simulink model "SarAdc"  (R2024a)
settings: Solver=VariableStepDiscrete  StartTime=0  StopTime=P.stop_time_s  RelTol=1e-3
PostLoadFcn:
  | addpath(genpath(fullfile(fileparts(fileparts(get_param(bdroot,'FileName'))),'src')),'-begin');
InitFcn:
  | addpath(genpath(fullfile(fileparts(fileparts(get_param(bdroot,'FileName'))),'src')),'-begin');
model workspace (MAT data in the model file):
  DecodeP.schema = 'sar20-behavior-decode/v1'
  DecodeP.vref_v = 5
  DecodeP.fsr_diff_v = 10
  DecodeP.ra_gain = 32
  DecodeP.d2_weights_ra_v = [0.36; 0.24; 0.16; 0.104; 0.064; 0.04; 0.024; 0.012; 0.008; 0.004; 0.002; 0.001]
  DecodeP.d2_offset_ra_v = -0.5095
  DecodeP.tracking_step_ra_v = 0.00025
  DecodeP.dither_enabled = 0
  DecodeP.dither_seed = 20261223
  DecodeP.dither_amplitude_v = 0.001
  DecodeP.calibration_mode = 'off'
  DecodeP.tracking_mode = 'finite_sinc2'
  DecodeP.az_mode = 'ordinary'
  DecodeP.coefficient_source = 'nominal saved.fpga weights only; new DAC1 geometry formula'
  DecodeP.d1_bias_v = 0
  P : object (value not decoded)
  TrainCaptureFile = ''
symbols that are objects in the model workspace (value not decoded): P
undefined symbols (not defined in the file): sar20_pp_initial_state, sar20_pp_verified_parameters
settings Model: Creator=Administrator  LastModifiedBy=Administrator
settings DataIOCC: SignalLogging=off

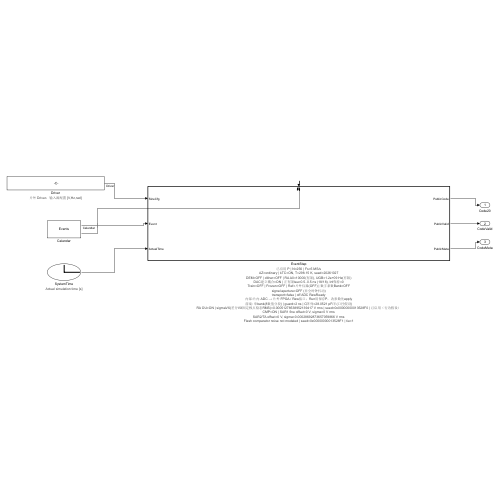
[thumbnail: Simulink's stored preview of the top-level diagram]
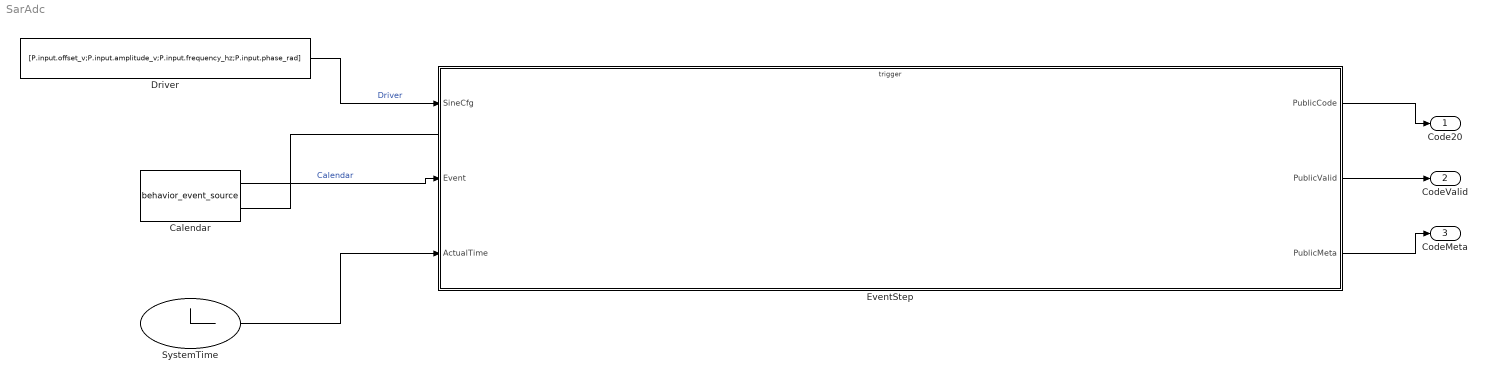
== system SarAdc ==
  Calendar : M-S-Function  FunctionName=behavior_event_source  Parameters=P.schedule
      mask Display: disp('Events')
  Driver : Constant  Value=[P.input.offset_v;P.input.amplitude_v;P.input.frequency_hz;P.input.phase_rad]
      settings: AttributesFormatString=片外 Driver：输入源配置 [V,Hz,rad]
  EventStep : Subsystem
      settings: AttributesFormatString=|
      | 已应用 P | N=256 | Fs=5 MS/s
      | AZ=ordinary | kTC=ON, T=298.15 K, seed=20261027
      | DEM=OFF | dither=OFF | RA A0=10000(有限), UGB=1.2e+09 Hz(有限)
      | DAC建立耦合=ON | 正有限tau=0.5..0.5 ns (18/18), Inf保持=0
      | Train=OFF | Frozen=OFF | Ref=片外仪器(OFF) | 数字系数Bank=OFF
      | signal aperture=OFF (非全时钟抖动)
      | transport=false | off ADC RawReady
      | 内部:片内 ADC → 片外 FPGA / Raw接口；Run用保存P，改参数先apply
      | 前端: 单bank(8数值分段) | guard=2 ns | C阵列=28.0521 pF/半(口径假设)
      | RA OU=ON | sigmaVX(差分VX固定极点稳态RMS)=0.00051278538952139417 V rms | seed=0x00000000013528F0 | 已启用（行为假设）
      | CMP=ON | SAR1 fine offset=0 V, sigma=0 V rms
      | SAR2/TA offset=0 V, sigma=0.00028692873657059866 V rms
      | Flash comparator noise not modeled | seed=0x00000000013528F1 | tie=1
  SystemTime : Clock
      settings: AttributesFormatString=Actual simulation time [s]
  Code20 : Outport  PortDimensions=1
  CodeValid : Outport  Port=2  PortDimensions=1
  CodeMeta : Outport  Port=3  PortDimensions=9
  wires:
  EventStep/3(PublicMeta) -> CodeMeta/1
  EventStep/2(PublicValid) -> CodeValid/1
  EventStep/1(PublicCode) -> Code20/1
  SystemTime/1 -> EventStep/3(ActualTime)
  Calendar/2 -> EventStep/Trigger
  Driver/1 -> EventStep/1(SineCfg)  "Driver"
  Calendar/1 -> EventStep/2(Event)  "Calendar"

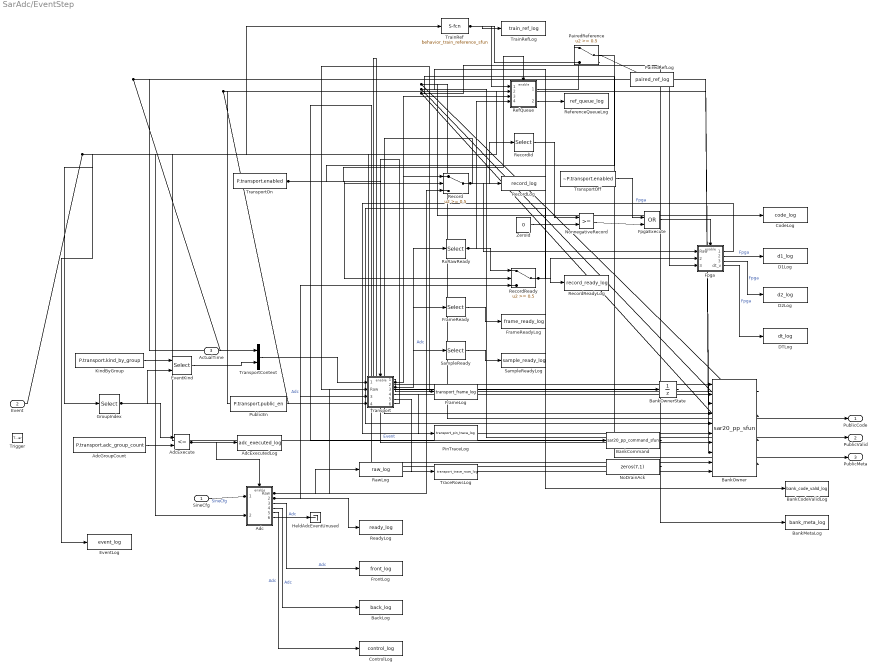
== system SarAdc/EventStep ==
  SineCfg : Inport  PortDimensions=4
  Event : Inport  Port=2  PortDimensions=2
  ActualTime : Inport  Port=3  PortDimensions=1
      settings: AttributesFormatString=Actual engine time [s] from root SystemTime
  Trigger : TriggerPort  TriggerType=either  VariantControl=(inherit)  ZeroCross=off  InitialTriggerSignalState=zero  PortDimensions=1
  Adc : Subsystem
      settings: AttributesFormatString=片内 ADC：Sample / DAC / RA-AZ / CT / SAR-Tracking
  AdcExecute : RelationalOperator  Operator=<=  OutDataTypeStr=boolean  RndMeth=Simplest  InputSameDT=off
  AdcExecutedLog : ToWorkspace  VariableName=adc_executed_log  SaveFormat=Timeseries  SampleTime=-1
  AdcGroupCount : Constant  Value=P.transport.adc_group_count
  BackLog : ToWorkspace  VariableName=back_log  SaveFormat=Timeseries  SampleTime=-1
  BankCodeValidLog : ToWorkspace  VariableName=bank_code_valid_log  SaveFormat=Timeseries  SampleTime=-1
  BankCommand : M-S-Function  FunctionName=sar20_pp_command_sfun  Parameters=sar20_pp_verified_parameters(P)
  BankMetaLog : ToWorkspace  VariableName=bank_meta_log  SaveFormat=Timeseries  SampleTime=-1
  BankOwner : M-S-Function  FunctionName=sar20_pp_sfun  Parameters=sar20_pp_verified_parameters(P)
  BankOwnerState : UnitDelay  InitialCondition=sar20_pp_initial_state(sar20_pp_verified_parameters(P))  SampleTime=-1  HasFrameUpgradeWarning=on
  CodeLog : ToWorkspace  VariableName=code_log  SaveFormat=Timeseries  SampleTime=-1
  ControlLog : ToWorkspace  VariableName=control_log  SaveFormat=Timeseries  SampleTime=-1
  D1Log : ToWorkspace  VariableName=d1_log  SaveFormat=Timeseries  SampleTime=-1
  D2Log : ToWorkspace  VariableName=d2_log  SaveFormat=Timeseries  SampleTime=-1
  DTLog : ToWorkspace  VariableName=dt_log  SaveFormat=Timeseries  SampleTime=-1
  EventKind : Selector  InputPortWidth=numel(P.groups)  IndexOptions=Index vector (port)  Indices=1  OutputSizes=1
  EventLog : ToWorkspace  VariableName=event_log  SaveFormat=Timeseries  SampleTime=-1
  Fpga : Subsystem
      settings: AttributesFormatString=片外 FPGA：公开Raw重构 | off ADC RawReady；开关显示不代表扫描覆盖
  FpgaExecute : Logic  Operator=OR  IconShape=distinctive  AllPortsSameDT=off  OutDataTypeStr=boolean
  FrameLog : ToWorkspace  VariableName=transport_frame_log  SaveFormat=Timeseries  SampleTime=-1
      settings: MaxDataPoints=P.transport.log_points
  FrameReady : Selector  Description=Transport.ready3(1)：完整接收帧脉冲，含startup VALID0帧与test槽。帧完成不代表有效ADC样本，不能用于参考查询或训练采集。  InputPortWidth=3  IndexOptions=Index vector (dialog)  Indices=1  OutputSizes=1
      settings: AttributesFormatString=|
      | 帧接收完成
      | 含startup/test
  FrameReadyLog : ToWorkspace  VariableName=frame_ready_log  SaveFormat=Timeseries  SampleTime=-1
      settings: MaxDataPoints=P.transport.log_points
  FrontLog : ToWorkspace  VariableName=front_log  SaveFormat=Timeseries  SampleTime=-1
  GroupIndex : Selector  InputPortWidth=2  IndexOptions=Index vector (dialog)  Indices=2  OutputSizes=1
  HeldAdcEventUnused : Terminator
  KindByGroup : Constant  Value=P.transport.kind_by_group
  NoDrainAck : Constant  Value=zeros(7,1)
  NonnegativeRecord : RelationalOperator  OutDataTypeStr=boolean  RndMeth=Simplest  InputSameDT=off
  PairedRefLog : ToWorkspace  VariableName=paired_ref_log  SaveFormat=Timeseries  SampleTime=-1
  PairedReference : Switch  Threshold=0.5  SaturateOnIntegerOverflow=off  InputSameDT=off
  PinTraceLog : ToWorkspace  VariableName=transport_pin_trace_log  SaveFormat=Timeseries  SampleTime=-1
      settings: MaxDataPoints=P.transport.trace_max_points
  PublicEn : Constant  Value=P.transport.public_en
  RawLog : ToWorkspace  VariableName=raw_log  SaveFormat=Timeseries  SampleTime=-1
  ReadyLog : ToWorkspace  VariableName=ready_log  SaveFormat=Timeseries  SampleTime=-1
  Record : Switch  Description=FPGA与训练/冻结支路的实际Raw6入口。OFF取ADC早期Raw；ON取公开pin-only RX。保留接收ID/epoch/valid，不改贴标签。startup负ID不执行FPGA解调。  Threshold=0.5  SaturateOnIntegerOverflow=off  InputSameDT=off
      settings: AttributesFormatString=|
      | FPGA实际Raw6
      | OFF ADC / ON RX
  RecordId : Selector  InputPortWidth=6  IndexOptions=Index vector (dialog)  Indices=4  OutputSizes=1
  RecordLog : ToWorkspace  VariableName=record_log  SaveFormat=Timeseries  SampleTime=-1
  RecordReady : Switch  Description=FPGA实际record_ready。OFF为ADC RawReady，ON为Transport.ready3(2)=raw_ready。不能替换为frame_ready或sample_ready；正常VALID0记录保留，由采集完整性门拒绝。  Threshold=0.5  SaturateOnIntegerOverflow=off  InputSameDT=off
      settings: AttributesFormatString=|
      | FPGA记录就绪
      | OFF ADC / ON raw_ready
  RecordReadyLog : ToWorkspace  VariableName=record_ready_log  SaveFormat=Timeseries  SampleTime=-1
  RefQueue : Subsystem  Description=片外外部仪器参考历史；只存TrainRef已公开的Ref4，按RX ID/epoch精确查询。不读ADC held/C/Qres，不计算第二份参考真值，也不向RX提供隐藏标签。仅raw_ready查询；OFF直接原TrainRef，ON提供同RX样本的历史参考。
      settings: AttributesFormatString=|
      | 片外参考历史对齐
      | 按RX ID/epoch查询
  ReferenceQueueLog : ToWorkspace  VariableName=ref_queue_log  SaveFormat=Timeseries  SampleTime=-1
      settings: MaxDataPoints=P.transport.log_points
  RxRawReady : Selector  Description=Transport.ready3(2)：RX正常非负ID、非test且无resync的RAW接收时点；仍可能VALID0。驱动record_ready与参考查询；无效记录由采集完整性门拒绝，不压缩日历。  InputPortWidth=3  IndexOptions=Index vector (dialog)  Indices=2  OutputSizes=1
      settings: AttributesFormatString=|
      | 正常RAW接收
      | 仍可能VALID0
  SampleReady : Selector  Description=Transport.ready3(3)=raw_ready AND ADC VALID。仅标有效样本诊断；不得用来静默删去无效训练槽。  InputPortWidth=3  IndexOptions=Index vector (dialog)  Indices=3  OutputSizes=1
      settings: AttributesFormatString=|
      | RAW且VALID
      | 有效样本诊断
  SampleReadyLog : ToWorkspace  VariableName=sample_ready_log  SaveFormat=Timeseries  SampleTime=-1
      settings: MaxDataPoints=P.transport.log_points
  TraceRowsLog : ToWorkspace  VariableName=transport_trace_rows_log  SaveFormat=Timeseries  SampleTime=-1
      settings: MaxDataPoints=P.transport.log_points
  TrainRef : M-S-Function  FunctionName=behavior_train_reference_sfun  Parameters=P.training.reference
      settings: AttributesFormatString=片外校准源参考 | V, ID, epoch, valid\nCNV锁存；理想参考假设；不读ADC节点
  TrainRefLog : ToWorkspace  VariableName=train_ref_log  SaveFormat=Timeseries  SampleTime=-1
      settings: MaxDataPoints=P.training.log_points
  Transport : Subsystem  Description=当前为片内TX与片外RX统一协议行为容器，尚未拆成两个可见子图。TX→公开pin事件→pin-only RX；接收标签由RX自行恢复，不传隐藏ID/epoch。32 bit，N−2流水；sample CNV到该样本RX完成为538 ns。+138 ns是当前slot相对CNV的close时刻，不是sample到RX总延迟。压缩事件行为不等于连续标量引脚波形，也不是LVDS电气或CDC签核。
      settings: AttributesFormatString=|
      | 片内TX / 片外RX（统一协议行为）
      | 32 bit | N−2 | sample→RX 538 ns
  TransportContext : Mux  Inputs=2
  TransportOff : Constant  Value=~P.transport.enabled
  TransportOn : Constant  Value=P.transport.enabled
  ZeroId : Constant  Value=0
  PublicCode : Outport  PortDimensions=1
  PublicValid : Outport  Port=2  PortDimensions=1
  PublicMeta : Outport  Port=3  PortDimensions=9
  wires:
  Adc/6(Event) -> HeldAdcEventUnused/1  "Adc"
  Adc/5(Control) -> ControlLog/1  "Adc"
  Adc/4(Backend) -> BackLog/1  "Adc"
  Adc/3(Frontend) -> FrontLog/1  "Adc"
  SineCfg/1 -> Adc/1(SineCfg)  "SineCfg"
  AdcExecute/1 -> AdcExecutedLog/1, Adc/Enable
  Adc/2(Ready) -> RecordReady/3, Transport/3(RawReady), ReadyLog/1  "Adc"
  Adc/1(Raw) -> Record/3, Transport/2(Raw), RawLog/1  "Adc"
  Fpga/2(d1_v) -> D1Log/1  "Fpga"
  Fpga/3(d2_v) -> D2Log/1  "Fpga"
  Fpga/4(dt_v) -> DTLog/1  "Fpga"
  GroupIndex/1 -> AdcExecute/1, EventKind/2
  AdcGroupCount/1 -> AdcExecute/2
  KindByGroup/1 -> EventKind/1
  EventKind/1 -> TransportContext/2
  TransportContext/1 -> Transport/1(Context)
  Transport/2(Ready3) -> FrameReady/1, RxRawReady/1, SampleReady/1
  Transport/1(RxRaw) -> Record/1, RefQueue/3(RxRaw)
  RxRawReady/1 -> RecordReady/1, RefQueue/4(RxReady)
  RecordId/1 -> NonnegativeRecord/1
  ZeroId/1 -> NonnegativeRecord/2
  TransportOff/1 -> FpgaExecute/1
  NonnegativeRecord/1 -> FpgaExecute/2
  FpgaExecute/1 -> Fpga/Enable
  FrameReady/1 -> FrameReadyLog/1
  SampleReady/1 -> SampleReadyLog/1
  Transport/3(Frame) -> FrameLog/1
  Transport/4(PinTrace) -> PinTraceLog/1
  Transport/5(TraceRows) -> TraceRowsLog/1
  RefQueue/2(QueueDiagnostic) -> ReferenceQueueLog/1
  BankOwner/4 -> BankMetaLog/1, PublicMeta/1
  BankOwner/3 -> BankCodeValidLog/1, PublicValid/1
  NoDrainAck/1 -> BankOwner/10
  BankCommand/1 -> BankOwner/9
  Transport/6(RxFault) -> BankOwner/7
  BankOwner/1 -> BankOwnerState/1
  BankOwnerState/1 -> BankOwner/1
  PairedReference/1 -> PairedRefLog/1, Fpga/3(TrainRef)
  RecordReady/1 -> BankOwner/5, RecordReadyLog/1, Fpga/2(RawReady)
  Record/1 -> BankOwner/4, RecordLog/1, RecordId/1, Fpga/1(Raw)
  RefQueue/1(PairedRef) -> PairedReference/1
  PublicEn/1 -> BankOwner/8, Transport/4(PublicEn)
  ActualTime/1 -> BankOwner/3, TransportContext/1
  TransportOn/1 -> PairedReference/2, RecordReady/2, Record/2, RefQueue/Enable, Transport/Enable
  Fpga/1(code20) -> BankOwner/6  "Fpga"
  TrainRef/1 -> PairedReference/3, RefQueue/1(Reference), TrainRefLog/1
  Event/1 -> BankCommand/1, BankOwner/2, TrainRef/1, Adc/2(Calendar), EventLog/1, GroupIndex/1, RefQueue/2(Event)  "Event"
  BankOwner/2 -> CodeLog/1, PublicCode/1

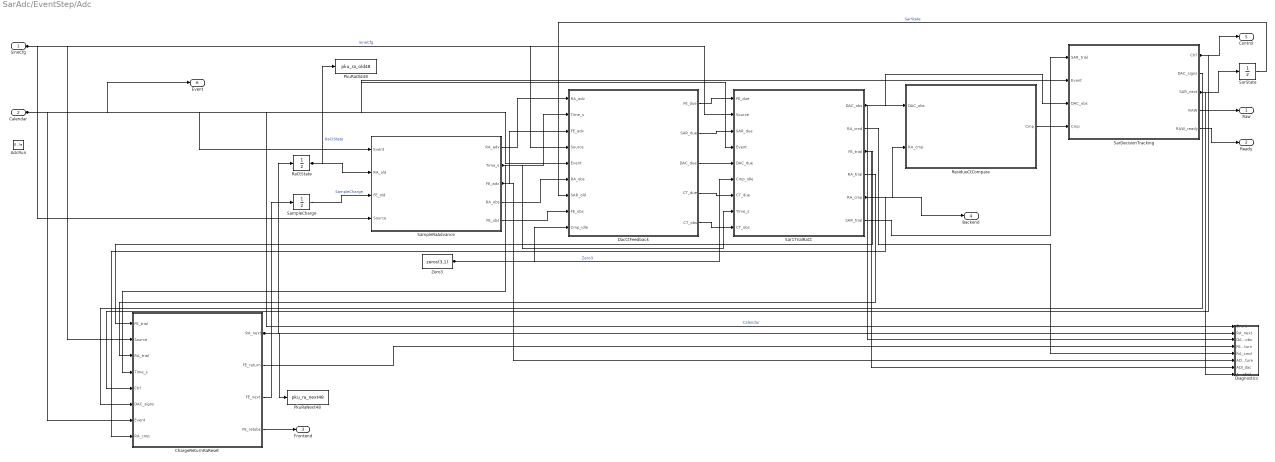
== system SarAdc/EventStep/Adc ==
  SineCfg : Inport  PortDimensions=4
  Calendar : Inport  Port=2  PortDimensions=2
  AdcRun : EnablePort
  ChargeReturnRaReset : Subsystem
  DacCtFeedback : Subsystem
  Diagnostics : Subsystem
  PkuRaNext48 : ToWorkspace  VariableName=pku_ra_next48  SaveFormat=Timeseries  SampleTime=-1
  PkuRaOld48 : ToWorkspace  VariableName=pku_ra_old48  SaveFormat=Timeseries  SampleTime=-1
  RaCtState : UnitDelay  InitialCondition=P.xBK0  SampleTime=-1  HasFrameUpgradeWarning=on
  ResidueCtCompare : Subsystem
  SampleCharge : UnitDelay  InitialCondition=P.xFE0  SampleTime=-1  HasFrameUpgradeWarning=on
  SampleRaAdvance : Subsystem
  Sar1TrialRaCt : Subsystem
  SarDecisionTracking : Subsystem
  SarState : UnitDelay  InitialCondition=P.xSC0  SampleTime=-1  HasFrameUpgradeWarning=on
  Zero3 : Constant  Value=zeros(3,1)
  Raw : Outport  PortDimensions=6
  Ready : Outport  Port=2  PortDimensions=1
  Frontend : Outport  Port=3  PortDimensions=7
  Backend : Outport  Port=4  PortDimensions=8
  Control : Outport  Port=5  PortDimensions=13
  Event : Outport  Port=6  PortDimensions=2
  wires:
  SineCfg/1 -> ChargeReturnRaReset/2(Source), DacCtFeedback/4(Source), Sar1TrialRaCt/2(Source), SampleRaAdvance/4(Source)  "SineCfg"
  SampleRaAdvance/1(RA_adv) -> DacCtFeedback/1(RA_adv)
  SampleRaAdvance/2(Time_s) -> DacCtFeedback/2(Time_s), Sar1TrialRaCt/8(Time_s), ChargeReturnRaReset/4(Time_s)
  DacCtFeedback/1(FE_due) -> Sar1TrialRaCt/1(FE_due)
  SampleRaAdvance/4(RA_obs) -> DacCtFeedback/6(RA_obs)
  SarState/1 -> DacCtFeedback/7(SAR_old)  "SarState"
  SampleRaAdvance/5(FE_obs) -> DacCtFeedback/8(FE_obs)
  Zero3/1 -> DacCtFeedback/9(Cmp_idle), Sar1TrialRaCt/6(Cmp_idle)  "Zero3"
  DacCtFeedback/2(SAR_due) -> Sar1TrialRaCt/3(SAR_due)
  DacCtFeedback/3(DAC_due) -> Sar1TrialRaCt/5(DAC_due)
  DacCtFeedback/4(CT_due) -> Sar1TrialRaCt/7(CT_due)
  Sar1TrialRaCt/4(RA_trial) -> ChargeReturnRaReset/3(RA_trial)
  SarDecisionTracking/1(Ctrl) -> ChargeReturnRaReset/5(Ctrl), Control/1
  SarDecisionTracking/2(DAC_signs) -> ChargeReturnRaReset/6(DAC_signs)
  Sar1TrialRaCt/5(RA_cmp) -> ChargeReturnRaReset/8(RA_cmp), ResidueCtCompare/2(RA_cmp), Backend/1
  SampleCharge/1 -> SampleRaAdvance/3(FE_old)  "SampleCharge"
  ChargeReturnRaReset/3(FE_next) -> SampleCharge/1
  Sar1TrialRaCt/6(SAR_trial) -> SarDecisionTracking/1(SAR_trial)
  ResidueCtCompare/1(Cmp) -> SarDecisionTracking/4(Cmp)
  DacCtFeedback/5(CT_obs) -> Sar1TrialRaCt/9(CT_obs)
  SarDecisionTracking/4(RAW) -> Raw/1
  SarDecisionTracking/5(RAW_ready) -> Ready/1
  ChargeReturnRaReset/4(FE_retobs) -> Frontend/1
  SarDecisionTracking/3(SAR_next) -> Diagnostics/8(ADI_control), SarState/1
  SampleRaAdvance/3(FE_adv) -> Diagnostics/6(ADI_capture), DacCtFeedback/3(FE_adv)
  Sar1TrialRaCt/3(FE_trial) -> Diagnostics/7(ADI_dac), ChargeReturnRaReset/1(FE_trial)
  Sar1TrialRaCt/2(RA_cmd) -> Diagnostics/5(RA_cmd)
  ChargeReturnRaReset/2(FE_return) -> Diagnostics/4(FE_return)
  Sar1TrialRaCt/1(DAC_obs) -> SarDecisionTracking/3(DAC_obs), ResidueCtCompare/1(DAC_obs), Diagnostics/3(DAC_obs)
  Calendar/1 -> SarDecisionTracking/2(Event), ChargeReturnRaReset/7(Event), Sar1TrialRaCt/4(Event), DacCtFeedback/5(Event), SampleRaAdvance/1(Event), Diagnostics/1(Event), Event/1  "Calendar"
  ChargeReturnRaReset/1(RA_next) -> PkuRaNext48/1, Diagnostics/2(RA_next), RaCtState/1
  RaCtState/1 -> PkuRaOld48/1, SampleRaAdvance/2(RA_old)  "RaCtState"

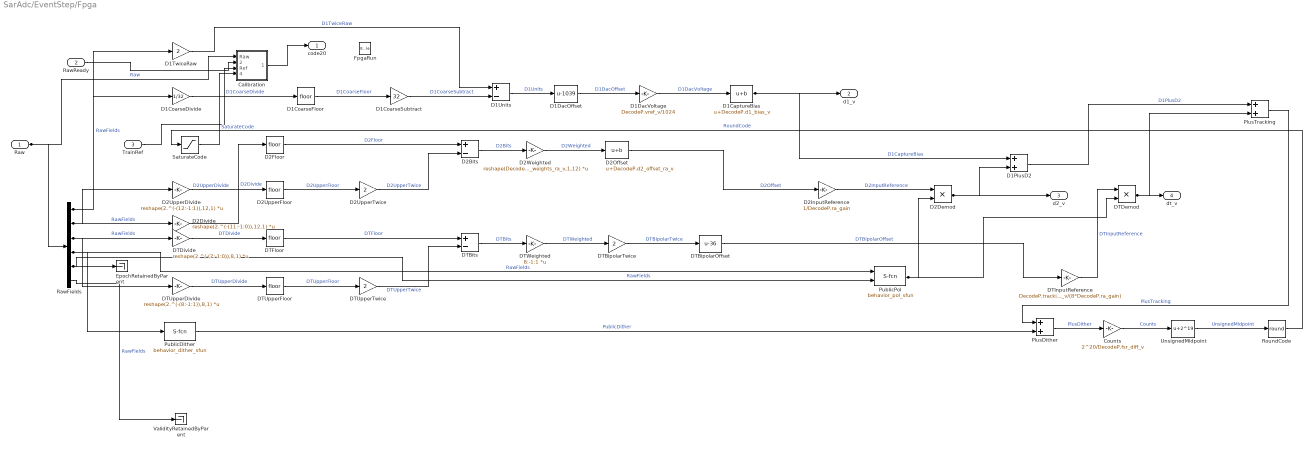
== system SarAdc/EventStep/Fpga ==
  Raw : Inport  PortDimensions=6
  RawReady : Inport  Port=2  PortDimensions=1
  TrainRef : Inport  Port=3  PortDimensions=4
  FpgaRun : EnablePort
  Calibration : Subsystem
  Counts : Gain  Gain=2^20/DecodeP.fsr_diff_v
  D1CaptureBias : Bias  Bias=DecodeP.d1_bias_v  SaturateOnIntegerOverflow=off
  D1CoarseDivide : Gain  Gain=1/32
  D1CoarseFloor : Rounding
  D1CoarseSubtract : Gain  Gain=32
  D1DacOffset : Bias  Bias=-1039  SaturateOnIntegerOverflow=off
  D1DacVoltage : Gain  Gain=DecodeP.vref_v/1024
  D1PlusD2 : Sum
  D1TwiceRaw : Gain  Gain=2
  D1Units : Sum  Inputs=+-
  D2Bits : Sum  Inputs=+-
  D2Demod : Product  Inputs=**
  D2Divide : Gain  Gain=reshape(2.^(-(11:-1:0)),12,1)  Multiplication=Matrix(K*u)
  D2Floor : Rounding
  D2InputReference : Gain  Gain=1/DecodeP.ra_gain
  D2Offset : Bias  Bias=DecodeP.d2_offset_ra_v  SaturateOnIntegerOverflow=off
  D2UpperDivide : Gain  Gain=reshape(2.^(-(12:-1:1)),12,1)  Multiplication=Matrix(K*u)
  D2UpperFloor : Rounding
  D2UpperTwice : Gain  Gain=2
  D2Weighted : Gain  Gain=reshape(DecodeP.d2_weights_ra_v,1,12)  Multiplication=Matrix(K*u)
  DTBipolarOffset : Bias  Bias=-36  SaturateOnIntegerOverflow=off
  DTBipolarTwice : Gain  Gain=2
  DTBits : Sum  Inputs=+-
  DTDemod : Product  Inputs=**
  DTDivide : Gain  Gain=reshape(2.^(-(7:-1:0)),8,1)  Multiplication=Matrix(K*u)
  DTFloor : Rounding
  DTInputReference : Gain  Gain=DecodeP.tracking_step_ra_v/(8*DecodeP.ra_gain)
  DTUpperDivide : Gain  Gain=reshape(2.^(-(8:-1:1)),8,1)  Multiplication=Matrix(K*u)
  DTUpperFloor : Rounding
  DTUpperTwice : Gain  Gain=2
  DTWeighted : Gain  Gain=8:-1:1  Multiplication=Matrix(K*u)
  EpochRetainedByParent : Terminator
  PlusDither : Sum
  PlusTracking : Sum
  PublicDither : M-S-Function  FunctionName=behavior_dither_sfun  Parameters=DecodeP
  PublicPol : M-S-Function  FunctionName=behavior_pol_sfun  Parameters=DecodeP
  RawFields : Demux  Outputs=6
  RoundCode : Rounding  Operator=round
  SaturateCode : Saturate  UpperLimit=2^20-1  LowerLimit=0
  UnsignedMidpoint : Bias  Bias=2^19  SaturateOnIntegerOverflow=off
  ValidityRetainedByParent : Terminator
  code20 : Outport  PortDimensions=1
  d1_v : Outport  Port=2  PortDimensions=1
  d2_v : Outport  Port=3  PortDimensions=1
  dt_v : Outport  Port=4  PortDimensions=1
  wires:
  DTUpperTwice/1 -> DTBits/2  "DTUpperTwice"
  DTFloor/1 -> DTBits/1  "DTFloor"
  DTUpperFloor/1 -> DTUpperTwice/1  "DTUpperFloor"
  DTUpperDivide/1 -> DTUpperFloor/1  "DTUpperDivide"
  DTDivide/1 -> DTFloor/1  "DTDivide"
  RawFields/3 -> DTUpperDivide/1, DTDivide/1  "RawFields"
  D2UpperTwice/1 -> D2Bits/2  "D2UpperTwice"
  D2Floor/1 -> D2Bits/1  "D2Floor"
  D2UpperFloor/1 -> D2UpperTwice/1  "D2UpperFloor"
  D2UpperDivide/1 -> D2UpperFloor/1  "D2UpperDivide"
  RawFields/6 -> ValidityRetainedByParent/1  "RawFields"
  DTBipolarTwice/1 -> DTBipolarOffset/1  "DTBipolarTwice"
  DTWeighted/1 -> DTBipolarTwice/1  "DTWeighted"
  DTBits/1 -> DTWeighted/1  "DTBits"
  D2Weighted/1 -> D2Offset/1  "D2Weighted"
  D2Bits/1 -> D2Weighted/1  "D2Bits"
  RawFields/1 -> D1TwiceRaw/1, D1CoarseDivide/1  "RawFields"
  DTInputReference/1 -> DTDemod/1  "DTInputReference"
  PublicPol/1 -> DTDemod/2, D2Demod/2
  D2InputReference/1 -> D2Demod/1  "D2InputReference"
  D2Offset/1 -> D2InputReference/1  "D2Offset"
  DTBipolarOffset/1 -> DTInputReference/1  "DTBipolarOffset"
  RawFields/4 -> PublicPol/1, PublicDither/1  "RawFields"
  RawFields/5 -> PublicPol/2, EpochRetainedByParent/1  "RawFields"
  Calibration/1(Code) -> code20/1
  SaturateCode/1 -> Calibration/4(NominalCode)  "SaturateCode"
  TrainRef/1 -> Calibration/3(Ref)
  RawReady/1 -> Calibration/2(Ready)
  PlusTracking/1 -> PlusDither/1  "PlusTracking"
  D1PlusD2/1 -> PlusTracking/1  "D1PlusD2"
  D1CaptureBias/1 -> d1_v/1, D1PlusD2/1  "D1CaptureBias"
  D2Demod/1 -> d2_v/1, D1PlusD2/2
  DTDemod/1 -> dt_v/1, PlusTracking/2
  Raw/1 -> Calibration/1(Raw), RawFields/1  "Raw"
  D1CoarseDivide/1 -> D1CoarseFloor/1  "D1CoarseDivide"
  D1CoarseFloor/1 -> D1CoarseSubtract/1  "D1CoarseFloor"
  D1TwiceRaw/1 -> D1Units/1  "D1TwiceRaw"
  D1CoarseSubtract/1 -> D1Units/2  "D1CoarseSubtract"
  D1Units/1 -> D1DacOffset/1  "D1Units"
  D1DacOffset/1 -> D1DacVoltage/1  "D1DacOffset"
  D1DacVoltage/1 -> D1CaptureBias/1  "D1DacVoltage"
  PublicDither/1 -> PlusDither/2  "PublicDither"
  PlusDither/1 -> Counts/1  "PlusDither"
  Counts/1 -> UnsignedMidpoint/1  "Counts"
  UnsignedMidpoint/1 -> RoundCode/1  "UnsignedMidpoint"
  RoundCode/1 -> SaturateCode/1  "RoundCode"
  RawFields/2 -> D2Divide/1, D2UpperDivide/1  "RawFields"
  D2Divide/1 -> D2Floor/1  "D2Divide"

== system SarAdc/EventStep/RefQueue ==
  Reference : Inport  PortDimensions=4
  Event : Inport  Port=2  PortDimensions=2
  RxRaw : Inport  Port=3  PortDimensions=6
  RxReady : Inport  Port=4  PortDimensions=1
  QueueRun : EnablePort
  ReferenceHistory : UnitDelay  InitialCondition=P.xREF0  SampleTime=-1  HasFrameUpgradeWarning=on
  ReferencePair : M-S-Function  FunctionName=behavior_reference_queue_sfun  Parameters=P.ref_queue
  PairedRef : Outport  PortDimensions=4
  QueueDiagnostic : Outport  Port=2  PortDimensions=4
  wires:
  ReferencePair/3 -> QueueDiagnostic/1
  ReferencePair/2 -> PairedRef/1
  RxReady/1 -> ReferencePair/5
  RxRaw/1 -> ReferencePair/4
  Event/1 -> ReferencePair/3
  Reference/1 -> ReferencePair/2
  ReferencePair/1 -> ReferenceHistory/1
  ReferenceHistory/1 -> ReferencePair/1

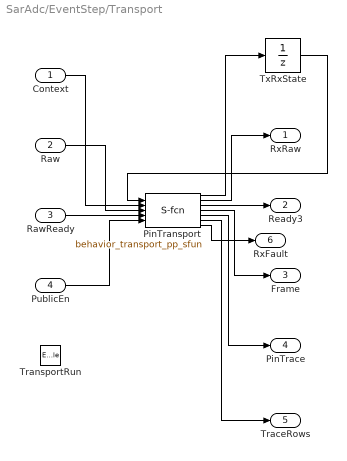
== system SarAdc/EventStep/Transport ==
  Context : Inport  PortDimensions=2
  Raw : Inport  Port=2  PortDimensions=6
  RawReady : Inport  Port=3  PortDimensions=1
  PublicEn : Inport  Port=4  PortDimensions=1
  TransportRun : EnablePort
  PinTransport : M-S-Function  FunctionName=behavior_transport_pp_sfun  Parameters=P.transport.core
  TxRxState : UnitDelay  InitialCondition=P.xTX0  SampleTime=-1  HasFrameUpgradeWarning=on
  RxRaw : Outport  PortDimensions=6
  Ready3 : Outport  Port=2  PortDimensions=3
  Frame : Outport  Port=3  PortDimensions=12
  PinTrace : Outport  Port=4  PortDimensions=[69 8]
  TraceRows : Outport  Port=5  PortDimensions=1  InitialOutput=0
  RxFault : Outport  Port=6  PortDimensions=1  InitialOutput=0
  wires:
  PinTransport/6 -> TraceRows/1
  PinTransport/5 -> PinTrace/1
  PinTransport/4 -> Frame/1
  PinTransport/3 -> Ready3/1
  PinTransport/2 -> RxRaw/1
  PublicEn/1 -> PinTransport/5
  RawReady/1 -> PinTransport/4
  Raw/1 -> PinTransport/3
  Context/1 -> PinTransport/2
  PinTransport/1 -> TxRxState/1
  TxRxState/1 -> PinTransport/1
  PinTransport/7 -> RxFault/1

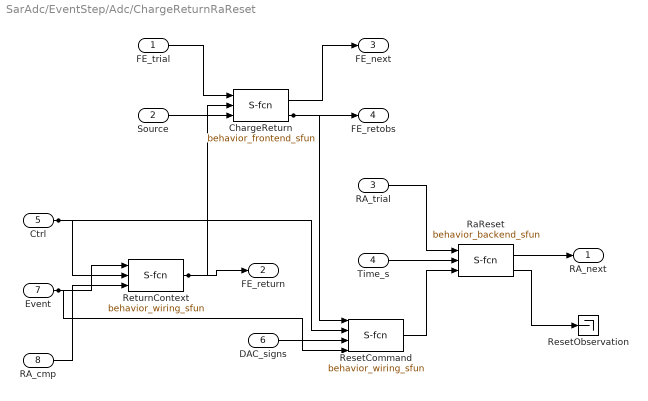
== system SarAdc/EventStep/Adc/ChargeReturnRaReset ==
  FE_trial : Inport  Description=Original source DacTrial.y1; 353 (legacy prefix 317 + aperture metadata 36) words; units packed mixed SI + tags; behavior_frontend_pack. Transparent boundary, no math/state.
  Source : Inport  Description=Original source SineCfg.y1; 4 words; units [V,V,Hz,rad]. Transparent boundary, no math/state.  Port=2
  RA_trial : Inport  Description=Original source RaAzCt.y1; 48 words; units packed mixed SI + command/tags; behavior_backend_pack. Transparent boundary, no math/state.  Port=3
  Time_s : Inport  Description=Original source Time.y1; 1 words; units s. Transparent boundary, no math/state.  Port=4
  Ctrl : Inport  Description=Original source Sar2Tracking.y2; 13 words; units [word,flags,RAW,tags,events]; behavior_control_stage. Transparent boundary, no math/state.  Port=5
  DAC_signs : Inport  Description=Original source Sar2Tracking.y3; 19 words; units 12 D2 + 7 TA signs. Transparent boundary, no math/state.  Port=6
  Event : Inport  Description=Original source Calendar.y1; 2 words; units [sample ID,group index]. Transparent boundary, no math/state.  Port=7
  RA_cmp : Inport  Description=Original source RaAzCt.y2; 8 words; units [V,V,V,V,1,s,V,V]. Transparent boundary, no math/state.  Port=8
  ChargeReturn : M-S-Function  FunctionName=behavior_frontend_sfun  Parameters='commit',P.front
  RaReset : M-S-Function  FunctionName=behavior_backend_sfun  Parameters='commit',P.backend
  ResetCommand : M-S-Function  FunctionName=behavior_wiring_sfun  Parameters='backend',P
  ResetObservation : Terminator
  ReturnContext : M-S-Function  FunctionName=behavior_wiring_sfun  Parameters='release',P
  RA_next : Outport  Description=Original source RaReset.y1; 48 words; units packed mixed SI + command/tags; behavior_backend_pack. Transparent boundary, no math/state.
  FE_return : Outport  Description=Original source ReturnContext.y1; 6 words; units [s,ID,epoch,event,D1,V]. Transparent boundary, no math/state.  Port=2
  FE_next : Outport  Description=Original source ChargeReturn.y1; 353 (legacy prefix 317 + aperture metadata 36) words; units packed mixed SI + tags; behavior_frontend_pack. Transparent boundary, no math/state.  Port=3
  FE_retobs : Outport  Description=Original source ChargeReturn.y2; 7 words; units [V,V,C,F,F,V,V]. Transparent boundary, no math/state.  Port=4
  wires:
  ChargeReturn/1 -> FE_next/1
  RaReset/1 -> RA_next/1
  RA_cmp/1 -> ReturnContext/3
  RaReset/2 -> ResetObservation/1
  Event/1 -> ReturnContext/1, ResetCommand/4
  DAC_signs/1 -> ResetCommand/3
  Ctrl/1 -> ReturnContext/2, ResetCommand/2
  ChargeReturn/2 -> FE_retobs/1, ResetCommand/1
  ResetCommand/1 -> RaReset/3
  Time_s/1 -> RaReset/2
  RA_trial/1 -> RaReset/1
  Source/1 -> ChargeReturn/3
  ReturnContext/1 -> FE_return/1, ChargeReturn/2
  FE_trial/1 -> ChargeReturn/1

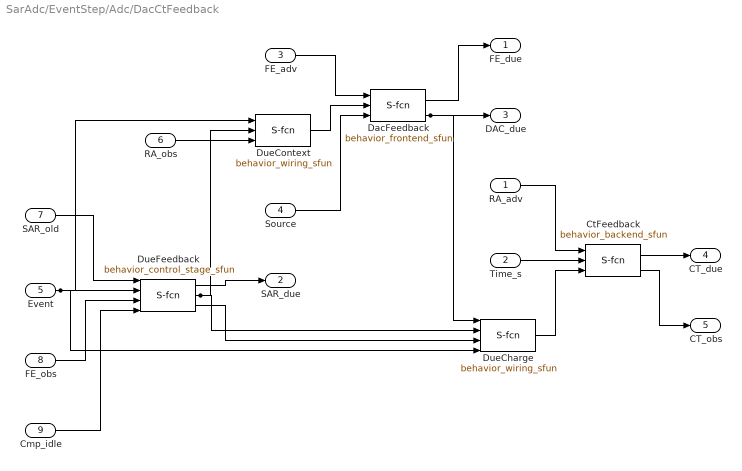
== system SarAdc/EventStep/Adc/DacCtFeedback ==
  RA_adv : Inport  Description=Original source RaAdvance.y1; 48 words; units packed mixed SI + command/tags; behavior_backend_pack. Transparent boundary, no math/state.
  Time_s : Inport  Description=Original source Time.y1; 1 words; units s. Transparent boundary, no math/state.  Port=2
  FE_adv : Inport  Description=Original source Sample.y1; 353 (legacy prefix 317 + aperture metadata 36) words; units packed mixed SI + tags; behavior_frontend_pack. Transparent boundary, no math/state.  Port=3
  Source : Inport  Description=Original source SineCfg.y1; 4 words; units [V,V,Hz,rad]. Transparent boundary, no math/state.  Port=4
  Event : Inport  Description=Original source Calendar.y1; 2 words; units [sample ID,group index]. Transparent boundary, no math/state.  Port=5
  RA_obs : Inport  Description=Original source RaAdvance.y2; 8 words; units [V,V,V,V,1,s,V,V]. Transparent boundary, no math/state.  Port=6
  SAR_old : Inport  Description=Original source SarState.y1; 51 words; units packed bits/counts/tags + sample V; behavior_sar_pack. Transparent boundary, no math/state.  Port=7
  FE_obs : Inport  Description=Original source Sample.y2; 7 words; units [V,V,C,F,F,V,V]. Transparent boundary, no math/state.  Port=8
  Cmp_idle : Inport  Description=Original source Zero3.y1; 3 words; units [decision,decision,V]. Transparent boundary, no math/state.  Port=9
  CtFeedback : M-S-Function  FunctionName=behavior_backend_sfun  Parameters='commit',P.backend
  DacFeedback : M-S-Function  FunctionName=behavior_frontend_sfun  Parameters='commit',P.front
  DueCharge : M-S-Function  FunctionName=behavior_wiring_sfun  Parameters='backend',P
  DueContext : M-S-Function  FunctionName=behavior_wiring_sfun  Parameters='due',P
  DueFeedback : M-S-Function  FunctionName=behavior_control_stage_sfun  Parameters='due',P
  FE_due : Outport  Description=Original source DacFeedback.y1; 353 (legacy prefix 317 + aperture metadata 36) words; units packed mixed SI + tags; behavior_frontend_pack. Transparent boundary, no math/state.
  SAR_due : Outport  Description=Original source DueFeedback.y1; 51 words; units packed bits/counts/tags + sample V; behavior_sar_pack. Transparent boundary, no math/state.  Port=2
  DAC_due : Outport  Description=Original source DacFeedback.y2; 7 words; units [V,V,C,F,F,V,V]. Transparent boundary, no math/state.  Port=3
  CT_due : Outport  Description=Original source CtFeedback.y1; 48 words; units packed mixed SI + command/tags; behavior_backend_pack. Transparent boundary, no math/state.  Port=4
  CT_obs : Outport  Description=Original source CtFeedback.y2; 8 words; units [V,V,V,V,1,s,V,V]. Transparent boundary, no math/state.  Port=5
  wires:
  CtFeedback/2 -> CT_obs/1
  CtFeedback/1 -> CT_due/1
  DueFeedback/1 -> SAR_due/1
  DacFeedback/1 -> FE_due/1
  Cmp_idle/1 -> DueFeedback/4
  FE_obs/1 -> DueFeedback/3
  SAR_old/1 -> DueFeedback/1
  RA_obs/1 -> DueContext/3
  Event/1 -> DueFeedback/2, DueContext/1, DueCharge/4
  DueFeedback/3 -> DueCharge/3
  DueFeedback/2 -> DueContext/2, DueCharge/2
  DacFeedback/2 -> DAC_due/1, DueCharge/1
  Source/1 -> DacFeedback/3
  DueContext/1 -> DacFeedback/2
  FE_adv/1 -> DacFeedback/1
  DueCharge/1 -> CtFeedback/3
  Time_s/1 -> CtFeedback/2
  RA_adv/1 -> CtFeedback/1

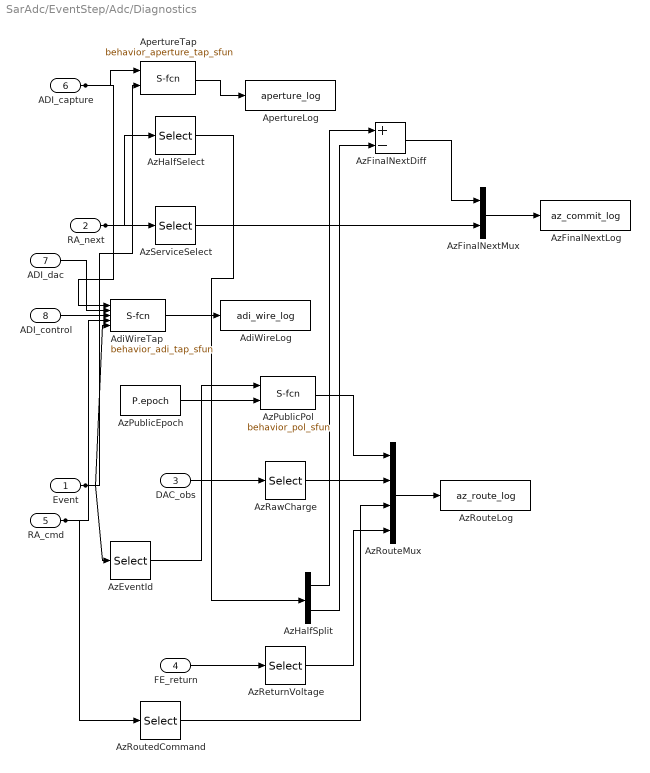
== system SarAdc/EventStep/Adc/Diagnostics ==
  Event : Inport  Description=Original source Calendar.y1; 2 words; units [sample ID,group index]. Transparent boundary, no math/state.
  RA_next : Inport  Description=Original source RaReset.y1; 48 words; units packed mixed SI + command/tags; behavior_backend_pack. Transparent boundary, no math/state.  Port=2
  DAC_obs : Inport  Description=Original source DacTrial.y2; 7 words; units [V,V,C,F,F,V,V]. Transparent boundary, no math/state.  Port=3
  FE_return : Inport  Description=Original source ReturnContext.y1; 6 words; units [s,ID,epoch,event,D1,V]. Transparent boundary, no math/state.  Port=4
  RA_cmd : Inport  Description=Original source RaCommand.y1; 26 words; units [C,F,19 signs,3 flags,ID,epoch]. Transparent boundary, no math/state.  Port=5
  ADI_capture : Inport  Port=6  PortDimensions=353
  ADI_dac : Inport  Port=7  PortDimensions=353
  ADI_control : Inport  Port=8  PortDimensions=51
  AdiWireLog : ToWorkspace  VariableName=adi_wire_log  SaveFormat=Timeseries  SampleTime=-1
      settings: MaxDataPoints=P.debug.adi_max_points
  AdiWireTap : M-S-Function  FunctionName=behavior_adi_tap_sfun  Parameters=P
  ApertureLog : ToWorkspace  VariableName=aperture_log  SaveFormat=Timeseries  SampleTime=-1
      settings: MaxDataPoints=P.debug.aperture_max_points
  ApertureTap : M-S-Function  FunctionName=behavior_aperture_tap_sfun  Parameters=P
  AzEventId : Selector  InputPortWidth=2  IndexOptions=Index vector (dialog)  Indices=1  OutputSizes=1
  AzFinalNextDiff : Sum  Inputs=+-
  AzFinalNextLog : ToWorkspace  VariableName=az_commit_log  SaveFormat=Timeseries  SampleTime=-1
  AzFinalNextMux : Mux  Inputs=2
  AzHalfSelect : Selector  InputPortWidth=48  IndexOptions=Index vector (dialog)  Indices=[3 4]  OutputSizes=2
  AzHalfSplit : Demux  Outputs=2
  AzPublicEpoch : Constant  Value=P.epoch
  AzPublicPol : M-S-Function  FunctionName=behavior_pol_sfun  Parameters=P.digital
  AzRawCharge : Selector  InputPortWidth=7  IndexOptions=Index vector (dialog)  Indices=3  OutputSizes=1
  AzReturnVoltage : Selector  InputPortWidth=6  IndexOptions=Index vector (dialog)  Indices=6  OutputSizes=1
  AzRouteLog : ToWorkspace  VariableName=az_route_log  SaveFormat=Timeseries  SampleTime=-1
  AzRouteMux : Mux
  AzRoutedCommand : Selector  InputPortWidth=26  IndexOptions=Index vector (dialog)  Indices=[1 22 23]  OutputSizes=3
  AzServiceSelect : Selector  InputPortWidth=48  IndexOptions=Index vector (dialog)  Indices=[38 39 40 41 42 43 48]  OutputSizes=7
  wires:
  AzReturnVoltage/1 -> AzRouteMux/4
  AzRawCharge/1 -> AzRouteMux/2
  AzPublicPol/1 -> AzRouteMux/1
  AzRouteMux/1 -> AzRouteLog/1
  FE_return/1 -> AzReturnVoltage/1
  DAC_obs/1 -> AzRawCharge/1
  AzPublicEpoch/1 -> AzPublicPol/2
  RA_next/1 -> AzServiceSelect/1, AzHalfSelect/1
  AzServiceSelect/1 -> AzFinalNextMux/2
  AzFinalNextDiff/1 -> AzFinalNextMux/1
  AzFinalNextMux/1 -> AzFinalNextLog/1
  AdiWireTap/1 -> AdiWireLog/1
  ADI_control/1 -> AdiWireTap/3
  ADI_dac/1 -> AdiWireTap/2
  AzEventId/1 -> AzPublicPol/1
  ApertureTap/1 -> ApertureLog/1
  RA_cmd/1 -> AzRoutedCommand/1, AdiWireTap/4
  Event/1 -> ApertureTap/2, AzEventId/1, AdiWireTap/5
  ADI_capture/1 -> ApertureTap/1, AdiWireTap/1
  AzHalfSplit/1 -> AzFinalNextDiff/1
  AzHalfSplit/2 -> AzFinalNextDiff/2
  AzHalfSelect/1 -> AzHalfSplit/1
  AzRoutedCommand/1 -> AzRouteMux/3

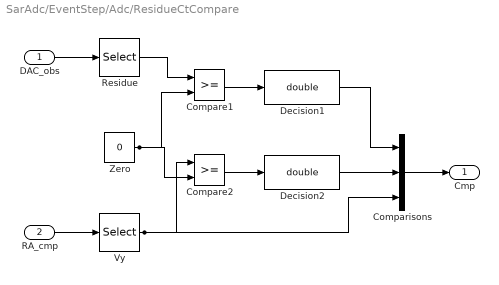
== system SarAdc/EventStep/Adc/ResidueCtCompare ==
  DAC_obs : Inport  Description=Original source DacTrial.y2; 7 words; units [V,V,C,F,F,V,V]. Transparent boundary, no math/state.
  RA_cmp : Inport  Description=Original source RaAzCt.y2; 8 words; units [V,V,V,V,1,s,V,V]. Transparent boundary, no math/state.  Port=2
  Compare1 : RelationalOperator  OutDataTypeStr=boolean  RndMeth=Simplest  InputSameDT=off
  Compare2 : RelationalOperator  OutDataTypeStr=boolean  RndMeth=Simplest  InputSameDT=off
  Comparisons : Mux  Inputs=3
  Decision1 : DataTypeConversion  OutDataTypeStr=double  SaturateOnIntegerOverflow=off  RndMeth=Floor
  Decision2 : DataTypeConversion  OutDataTypeStr=double  SaturateOnIntegerOverflow=off  RndMeth=Floor
  Residue : Selector  InputPortWidth=7  IndexOptions=Index vector (dialog)  Indices=2  OutputSizes=1
  Vy : Selector  InputPortWidth=8  IndexOptions=Index vector (dialog)  Indices=2  OutputSizes=1
  Zero : Constant  Value=0
  Cmp : Outport  Description=Original source Comparisons.y1; 3 words; units [decision,decision,V]. Transparent boundary, no math/state.
  wires:
  Comparisons/1 -> Cmp/1
  RA_cmp/1 -> Vy/1
  DAC_obs/1 -> Residue/1
  Compare2/1 -> Decision2/1
  Compare1/1 -> Decision1/1
  Decision2/1 -> Comparisons/2
  Decision1/1 -> Comparisons/1
  Vy/1 -> Comparisons/3, Compare2/1
  Zero/1 -> Compare2/2, Compare1/2
  Residue/1 -> Compare1/1

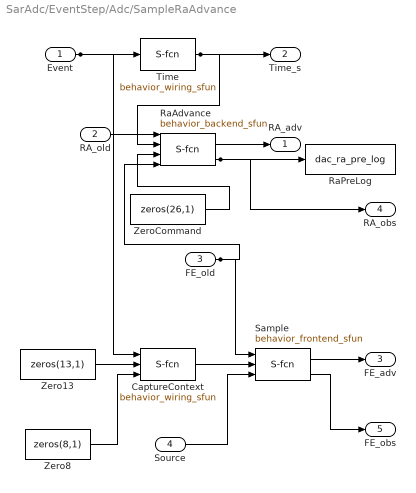
== system SarAdc/EventStep/Adc/SampleRaAdvance ==
  Event : Inport  Description=Original source Calendar.y1; 2 words; units [sample ID,group index]. Transparent boundary, no math/state.
  RA_old : Inport  Description=Original source RaCtState.y1; 48 words; units packed mixed SI + command/tags; behavior_backend_pack. Transparent boundary, no math/state.  Port=2
  FE_old : Inport  Description=Original source SampleCharge.y1; 353 (legacy prefix 317 + aperture metadata 36) words; units packed mixed SI + tags; behavior_frontend_pack. Transparent boundary, no math/state.  Port=3
  Source : Inport  Description=Original source SineCfg.y1; 4 words; units [V,V,Hz,rad]. Transparent boundary, no math/state.  Port=4
  CaptureContext : M-S-Function  FunctionName=behavior_wiring_sfun  Parameters='cnv',P
  RaAdvance : M-S-Function  FunctionName=behavior_backend_sfun  Parameters='advance',behavior_dac_backend_parameters(P)
  RaPreLog : ToWorkspace  VariableName=dac_ra_pre_log  SaveFormat=Timeseries  SampleTime=-1
      settings: Description=Actual RaAdvance.y2 obs8 before CINC feedback/kick and command commit; not BackLog.  MaxDataPoints=P.debug.dac_max_points
  Sample : M-S-Function  FunctionName=behavior_frontend_sfun  Parameters='advance',P.front
  Time : M-S-Function  FunctionName=behavior_wiring_sfun  Parameters='clock',P
  Zero13 : Constant  Value=zeros(13,1)
  Zero8 : Constant  Value=zeros(8,1)
  ZeroCommand : Constant  Value=zeros(26,1)
  RA_adv : Outport  Description=Original source RaAdvance.y1; 48 words; units packed mixed SI + command/tags; behavior_backend_pack. Transparent boundary, no math/state.
  Time_s : Outport  Description=Original source Time.y1; 1 words; units s. Transparent boundary, no math/state.  Port=2
  FE_adv : Outport  Description=Original source Sample.y1; 353 (legacy prefix 317 + aperture metadata 36) words; units packed mixed SI + tags; behavior_frontend_pack. Transparent boundary, no math/state.  Port=3
  RA_obs : Outport  Description=Original source RaAdvance.y2; 8 words; units [V,V,V,V,1,s,V,V]. Transparent boundary, no math/state.  Port=4
  FE_obs : Outport  Description=Original source Sample.y2; 7 words; units [V,V,C,F,F,V,V]. Transparent boundary, no math/state.  Port=5
  wires:
  Sample/2 -> FE_obs/1
  Sample/1 -> FE_adv/1
  Source/1 -> Sample/3
  CaptureContext/1 -> Sample/2
  Zero8/1 -> CaptureContext/3
  Zero13/1 -> CaptureContext/2
  Event/1 -> Time/1, CaptureContext/1
  FE_old/1 -> Sample/1, RaAdvance/4
  RA_old/1 -> RaAdvance/1
  Time/1 -> RaAdvance/2, Time_s/1
  ZeroCommand/1 -> RaAdvance/3
  RaAdvance/1 -> RA_adv/1
  RaAdvance/2 -> RaPreLog/1, RA_obs/1

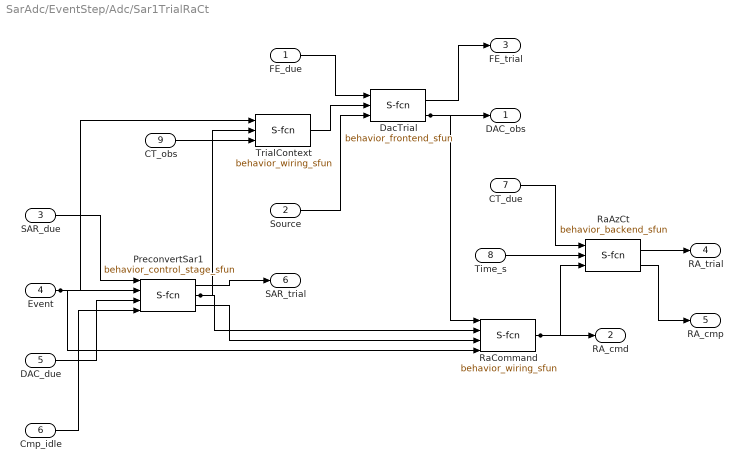
== system SarAdc/EventStep/Adc/Sar1TrialRaCt ==
  FE_due : Inport  Description=Original source DacFeedback.y1; 353 (legacy prefix 317 + aperture metadata 36) words; units packed mixed SI + tags; behavior_frontend_pack. Transparent boundary, no math/state.
  Source : Inport  Description=Original source SineCfg.y1; 4 words; units [V,V,Hz,rad]. Transparent boundary, no math/state.  Port=2
  SAR_due : Inport  Description=Original source DueFeedback.y1; 51 words; units packed bits/counts/tags + sample V; behavior_sar_pack. Transparent boundary, no math/state.  Port=3
  Event : Inport  Description=Original source Calendar.y1; 2 words; units [sample ID,group index]. Transparent boundary, no math/state.  Port=4
  DAC_due : Inport  Description=Original source DacFeedback.y2; 7 words; units [V,V,C,F,F,V,V]. Transparent boundary, no math/state.  Port=5
  Cmp_idle : Inport  Description=Original source Zero3.y1; 3 words; units [decision,decision,V]. Transparent boundary, no math/state.  Port=6
  CT_due : Inport  Description=Original source CtFeedback.y1; 48 words; units packed mixed SI + command/tags; behavior_backend_pack. Transparent boundary, no math/state.  Port=7
  Time_s : Inport  Description=Original source Time.y1; 1 words; units s. Transparent boundary, no math/state.  Port=8
  CT_obs : Inport  Description=Original source CtFeedback.y2; 8 words; units [V,V,V,V,1,s,V,V]. Transparent boundary, no math/state.  Port=9
  DacTrial : M-S-Function  FunctionName=behavior_frontend_sfun  Parameters='commit',P.front
  PreconvertSar1 : M-S-Function  FunctionName=behavior_control_stage_sfun  Parameters='prepare',P
  RaAzCt : M-S-Function  FunctionName=behavior_backend_sfun  Parameters='commit',P.backend
  RaCommand : M-S-Function  FunctionName=behavior_wiring_sfun  Parameters='backend',P
  TrialContext : M-S-Function  FunctionName=behavior_wiring_sfun  Parameters='trial',P
  DAC_obs : Outport  Description=Original source DacTrial.y2; 7 words; units [V,V,C,F,F,V,V]. Transparent boundary, no math/state.
  RA_cmd : Outport  Description=Original source RaCommand.y1; 26 words; units [C,F,19 signs,3 flags,ID,epoch]. Transparent boundary, no math/state.  Port=2
  FE_trial : Outport  Description=Original source DacTrial.y1; 353 (legacy prefix 317 + aperture metadata 36) words; units packed mixed SI + tags; behavior_frontend_pack. Transparent boundary, no math/state.  Port=3
  RA_trial : Outport  Description=Original source RaAzCt.y1; 48 words; units packed mixed SI + command/tags; behavior_backend_pack. Transparent boundary, no math/state.  Port=4
  RA_cmp : Outport  Description=Original source RaAzCt.y2; 8 words; units [V,V,V,V,1,s,V,V]. Transparent boundary, no math/state.  Port=5
  SAR_trial : Outport  Description=Original source PreconvertSar1.y1; 51 words; units packed bits/counts/tags + sample V; behavior_sar_pack. Transparent boundary, no math/state.  Port=6
  wires:
  PreconvertSar1/1 -> SAR_trial/1
  RaAzCt/2 -> RA_cmp/1
  RaAzCt/1 -> RA_trial/1
  DacTrial/1 -> FE_trial/1
  CT_obs/1 -> TrialContext/3
  PreconvertSar1/3 -> RaCommand/3
  PreconvertSar1/2 -> TrialContext/2, RaCommand/2
  DacTrial/2 -> DAC_obs/1, RaCommand/1
  RaCommand/1 -> RA_cmd/1, RaAzCt/3
  Time_s/1 -> RaAzCt/2
  CT_due/1 -> RaAzCt/1
  Cmp_idle/1 -> PreconvertSar1/4
  DAC_due/1 -> PreconvertSar1/3
  Event/1 -> TrialContext/1, RaCommand/4, PreconvertSar1/2
  SAR_due/1 -> PreconvertSar1/1
  Source/1 -> DacTrial/3
  TrialContext/1 -> DacTrial/2
  FE_due/1 -> DacTrial/1

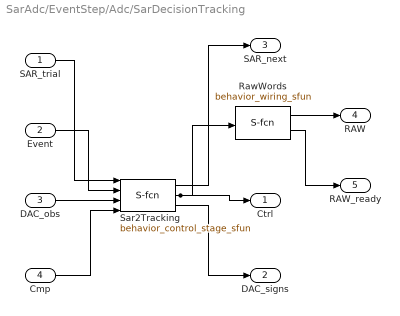
== system SarAdc/EventStep/Adc/SarDecisionTracking ==
  SAR_trial : Inport  Description=Original source PreconvertSar1.y1; 51 words; units packed bits/counts/tags + sample V; behavior_sar_pack. Transparent boundary, no math/state.
  Event : Inport  Description=Original source Calendar.y1; 2 words; units [sample ID,group index]. Transparent boundary, no math/state.  Port=2
  DAC_obs : Inport  Description=Original source DacTrial.y2; 7 words; units [V,V,C,F,F,V,V]. Transparent boundary, no math/state.  Port=3
  Cmp : Inport  Description=Original source Comparisons.y1; 3 words; units [decision,decision,V]. Transparent boundary, no math/state.  Port=4
  RawWords : M-S-Function  FunctionName=behavior_wiring_sfun  Parameters='raw',P
  Sar2Tracking : M-S-Function  FunctionName=behavior_control_stage_sfun  Parameters='decide',P
  Ctrl : Outport  Description=Original source Sar2Tracking.y2; 13 words; units [word,flags,RAW,tags,events]; behavior_control_stage. Transparent boundary, no math/state.
  DAC_signs : Outport  Description=Original source Sar2Tracking.y3; 19 words; units 12 D2 + 7 TA signs. Transparent boundary, no math/state.  Port=2
  SAR_next : Outport  Description=Original source Sar2Tracking.y1; 51 words; units packed bits/counts/tags + sample V; behavior_sar_pack. Transparent boundary, no math/state.  Port=3
  RAW : Outport  Description=Original source RawWords.y1; 6 words; units [D1,D2,DT,ID,epoch,valid]. Transparent boundary, no math/state.  Port=4
  RAW_ready : Outport  Description=Original source RawWords.y2; 1 words; units boolean. Transparent boundary, no math/state.  Port=5
  wires:
  RawWords/2 -> RAW_ready/1
  RawWords/1 -> RAW/1
  Sar2Tracking/1 -> SAR_next/1
  Sar2Tracking/3 -> DAC_signs/1
  Cmp/1 -> Sar2Tracking/4
  DAC_obs/1 -> Sar2Tracking/3
  Event/1 -> Sar2Tracking/2
  SAR_trial/1 -> Sar2Tracking/1
  Sar2Tracking/2 -> Ctrl/1, RawWords/1

== system SarAdc/EventStep/Fpga/Calibration ==
  Raw : Inport  PortDimensions=6
  Ready : Inport  Port=2  PortDimensions=1
  Ref : Inport  Port=3  PortDimensions=4
  NominalCode : Inport  Port=4  PortDimensions=1
  CalStatus : ToWorkspace  VariableName=cal_status_log  SaveFormat=Timeseries  SampleTime=-1
      settings: MaxDataPoints=1
  FitSnapshot : ToWorkspace  VariableName=cal_fit_log  SaveFormat=Timeseries  SampleTime=-1
      settings: MaxDataPoints=1
  FrozenDecode : M-S-Function  FunctionName=behavior_frozen_sfun  Parameters=P.frozen.enabled,P.frozen.cache
      settings: AttributesFormatString=|
      | FPGA固定系数重构 | RAW/Ready
      | 不接Ref，不训练；冻结候选用于独立holdout
  FrozenLog : ToWorkspace  VariableName=frozen_log  SaveFormat=Timeseries  SampleTime=-1
      settings: MaxDataPoints=P.frozen.log_points
  NominalLog : ToWorkspace  VariableName=nominal_code_log  SaveFormat=Timeseries  SampleTime=-1
      settings: MaxDataPoints=P.frozen.log_points
  Train : M-S-Function  FunctionName=behavior_cal_train_sfun  Parameters=P.cal_cfg,TrainCaptureFile
      settings: AttributesFormatString=FPGA/PC训练收集 | 公开RAW + 外部Ref\nUpdate收帧/拟合；Code保持名义输出；不自动冻结
  Code : Outport
  wires:
  FrozenDecode/2 -> FrozenLog/1
  FrozenDecode/1 -> Code/1
  Raw/1 -> FrozenDecode/1, Train/1
  Ready/1 -> FrozenDecode/2, Train/2
  Ref/1 -> Train/3
  NominalCode/1 -> Train/4
  Train/2 -> CalStatus/1
  Train/3 -> FitSnapshot/1
  Train/1 -> NominalLog/1, FrozenDecode/3
